simulink model "USV_MultiWaypoints"  (R2026b)
settings: Solver=VariableStepAuto  StopTime=300
undefined symbols (not defined in the file): arrival_dwell_time, arrival_radius, arrival_speed, current_bias_x, current_bias_y, current_change_time, current_estimation_tau, current_x, drag_r, drag_u, F_max, inertia_z, integral_activation_radius, K_aw, K_distance, Kd_heading, Ki_position, Ki_u, Kp_heading, Kp_u, M_max, mass_usv, position_integral_limit, u_max, wp1_x, wp1_y, wp2_x, wp2_y, wp3_x, wp3_y
libraries: simulink x1
settings Model: Creator=pablo  LastModifiedBy=pablo

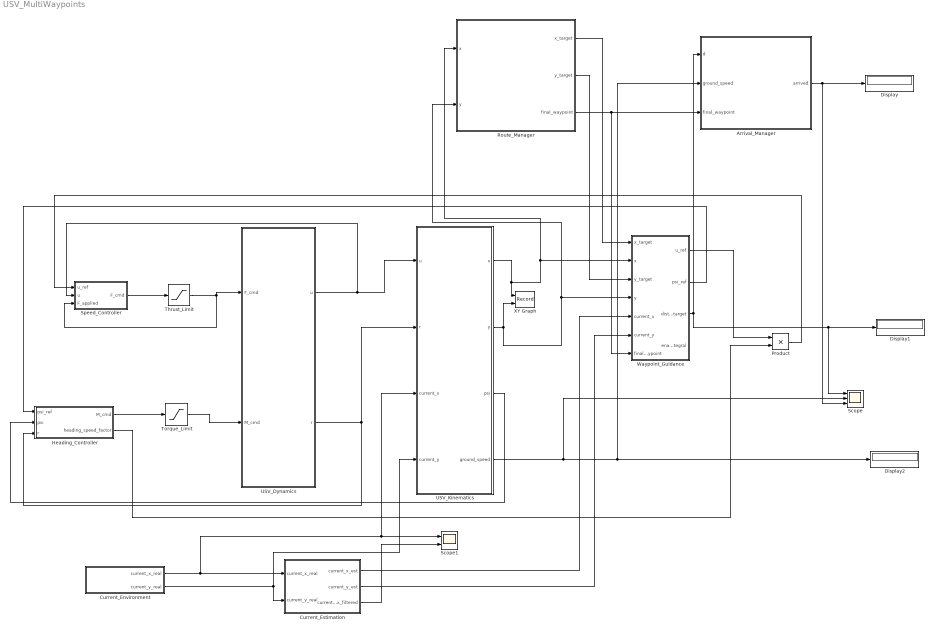
== system USV_MultiWaypoints ==
  Arrival_Manager : Stateflow chart  TreatAsAtomicUnit=on
  Current_Environment : Subsystem
  Current_Estimation : Subsystem
  Display : Display
  Display1 : Display
  Display2 : Display
  Heading_Controller : Subsystem
  Product : Product
  Route_Manager : Stateflow chart  TreatAsAtomicUnit=on
  Scope : Scope  NumInputPorts=3
      settings: ActiveDisplayYMinimum=-3.9141031212329302  ActiveDisplayYMaximum=39.009126348576444
  Scope1 : Scope  NumInputPorts=2
      settings: ActiveDisplayYMinimum=-0.25  ActiveDisplayYMaximum=0.25
  Speed_Controller : Subsystem
  Thrust_Limit : Saturate  UpperLimit=F_max  LowerLimit=-F_max
  Torque_Limit : Saturate  UpperLimit=M_max  LowerLimit=-M_max
  USV_Dynamics : Subsystem
  USV_Kinematics : Subsystem
  Waypoint_Guidance : Subsystem
  XY Graph : Record  NumPorts=2.0  FileSettingsInternal="{\"entries\":[{\"content\":{\"excelSettings\":{\"content\":{},\"type\":\"Streamout.ExcelSettings\"},\"parquetSettings\":{\"content\":{},\"type\":\"Streamout.ParquetSettings\"}},\"type\":\"Streamout.FileSettingStorage\",\"uuid\":\"\"}],\"packageUris\":[\"http:\\/\\/schema.mathworks.com\\/mf0\\/streamout_blocks\\/R2020a\"],\"version\":\"1.0\"}"  FrameSettings=[0, 0]  Layout=[1 1]  SignalsInternal="{\"entries\":[{\"content\":{\"signals\":[{\"content\":{\"blockPath\":[],\"dimensions\":[1],\"domain\":\"\",\"lineColor\":\"#a2142f\",\"plots\":[ 1 ],\"port\":1,\"sid\":[\"\"],\"signalID\":1,\"signalName\":\"USV_Kinematics:1\"},\"type\":\"RecordBlkView.Signal\",\"uuid\":\"\"},{\"content\":{\"blockPath\":[],\"dimensions\":[1],\"domain\":\"\",\"lineColor\":\"#139fff\",\"plots\":[ 1 ],\"port\":2,\"sid\":[\"\"],\"signalID\":2,\"signalName\":\"USV_Kinematics:2\"},\"type\":\"RecordBlkView.Signal\",\"uuid\":\"\"}]},\"type\":\"RecordBlkView.InputSignals\",\"uuid\":\"\"}],\"packageUris\":[\"http:\\/\\/schema.mathworks.com\\/mf0\\/streamout_blocks\\/R2020a\"],\"version\":\"1.0\"}"  VisualizationBindings="{\"xyplotplugin\":{\"info\":[{\"series\":[{\"bindingParametersList\":[{\"parameter\":\"X-Axis\",\"signalID\":1,\"signalName\":\"USV_Kinematics:1\"},{\"parameter\":\"Y-Axis\",\"signalID\":2,\"signalName\":\"USV_Kinematics:2\"}],\"seriesID\":0}],\"subplotID\":1}]}}"  CompatibilityTag=XY
  wires:
  USV_Dynamics/1(u) -> Speed_Controller/2(u), USV_Kinematics/1(u)
  USV_Dynamics/2(r) -> Heading_Controller/3(r), USV_Kinematics/2(r)
  Speed_Controller/1(F_cmd) -> Thrust_Limit/1
  Heading_Controller/1(M_cmd) -> Torque_Limit/1
  USV_Kinematics/3(psi) -> Heading_Controller/2(psi)
  USV_Kinematics/1(x) -> XY Graph/1, Route_Manager/1(x), Waypoint_Guidance/2(x)
  USV_Kinematics/2(y) -> Route_Manager/2(y), Waypoint_Guidance/4(y), XY Graph/2
  Waypoint_Guidance/2(psi_ref) -> Heading_Controller/1(psi_ref)
  Waypoint_Guidance/1(u_ref) -> Product/1
  Arrival_Manager/1(arrived) -> Scope/3, Display/1
  Waypoint_Guidance/3(distance_to_target) -> Arrival_Manager/1(d), Scope/1, Display1/1
  Route_Manager/1(x_target) -> Waypoint_Guidance/1(x_target)
  Route_Manager/2(y_target) -> Waypoint_Guidance/3(y_target)
  Route_Manager/3(final_waypoint) -> Waypoint_Guidance/7(final_waypoint), Arrival_Manager/3(final_waypoint)
  Thrust_Limit/1 -> USV_Dynamics/1(F_cmd), Speed_Controller/3(F_applied)
  Torque_Limit/1 -> USV_Dynamics/2(M_cmd)
  Heading_Controller/2(heading_speed_factor) -> Product/2
  Product/1 -> Speed_Controller/1(u_ref)
  USV_Kinematics/4(ground_speed) -> Scope/2, Arrival_Manager/2(ground_speed), Display2/1
  Current_Estimation/1(current_x_est) -> Waypoint_Guidance/5(current_x)
  Current_Estimation/2(current_y_est) -> Waypoint_Guidance/6(current_y)
  Current_Estimation/3(current_x_filtered) -> Scope1/2
  Current_Environment/1(current_x_real) -> Scope1/1, USV_Kinematics/3(current_x), Current_Estimation/1(current_x_real)
  Current_Environment/2(current_y_real) -> Current_Estimation/2(current_y_real), USV_Kinematics/4(current_y)

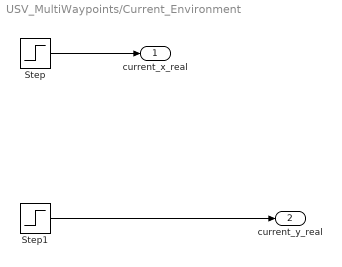
== system USV_MultiWaypoints/Current_Environment ==
  Step : Step  Time=current_change_time  InitialValue=current_x  FinalValue=current_x_after  SampleTime=0
  Step1 : Step  Time=current_change_time  InitialValue=current_y  FinalValue=current_y_after  SampleTime=0
  current_x_real : Outport
  current_y_real : Outport  Port=2
  wires:
  Step/1 -> current_x_real/1
  Step1/1 -> current_y_real/1

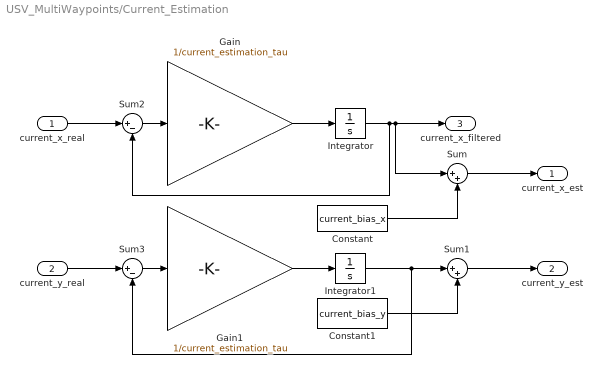
== system USV_MultiWaypoints/Current_Estimation ==
  current_x_real : Inport
  current_y_real : Inport  Port=2
  Constant : Constant  Value=current_bias_x
  Constant1 : Constant  Value=current_bias_y
  Gain : Gain  Gain=1/current_estimation_tau
  Gain1 : Gain  Gain=1/current_estimation_tau
  Integrator : Integrator  InitialCondition=current_x
  Integrator1 : Integrator  InitialCondition=current_x
  Sum : Sum  Inputs=|++
  Sum1 : Sum  Inputs=|++
  Sum2 : Sum  Inputs=|+-
  Sum3 : Sum  Inputs=|+-
  current_x_est : Outport
  current_y_est : Outport  Port=2
  current_x_filtered : Outport  Port=3
  wires:
  current_y_real/1 -> Sum3/1
  current_x_real/1 -> Sum2/1
  Gain1/1 -> Integrator1/1
  Sum2/1 -> Gain/1
  Sum3/1 -> Gain1/1
  Gain/1 -> Integrator/1
  Integrator/1 -> Sum/1, current_x_filtered/1, Sum2/2
  Constant/1 -> Sum/2
  Integrator1/1 -> Sum3/2, Sum1/1
  Constant1/1 -> Sum1/2
  Sum/1 -> current_x_est/1
  Sum1/1 -> current_y_est/1

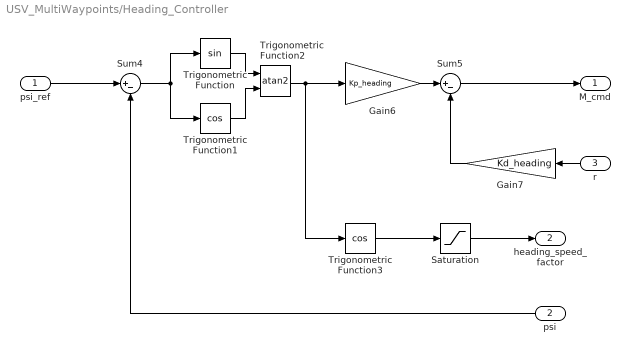
== system USV_MultiWaypoints/Heading_Controller ==
  psi_ref : Inport
  psi : Inport  Port=2
  r : Inport  Port=3
  Gain6 : Gain  Gain=Kp_heading
  Gain7 : Gain  Gain=Kd_heading
  Saturation : Saturate  UpperLimit=1  LowerLimit=0
  Sum4 : Sum  Inputs=|+-
  Sum5 : Sum  Inputs=|+-
  Trigonometric Function : Trigonometry
  Trigonometric Function1 : Trigonometry  Operator=cos
  Trigonometric Function2 : Trigonometry  Operator=atan2
  Trigonometric Function3 : Trigonometry  Operator=cos
  M_cmd : Outport
  heading_speed_factor : Outport  Port=2
  wires:
  Sum5/1 -> M_cmd/1
  psi_ref/1 -> Sum4/1
  r/1 -> Gain7/1
  Gain6/1 -> Sum5/1
  psi/1 -> Sum4/2
  Gain7/1 -> Sum5/2
  Sum4/1 -> Trigonometric Function/1, Trigonometric Function1/1
  Trigonometric Function/1 -> Trigonometric Function2/1
  Trigonometric Function1/1 -> Trigonometric Function2/2
  Trigonometric Function2/1 -> Trigonometric Function3/1, Gain6/1
  Trigonometric Function3/1 -> Saturation/1
  Saturation/1 -> heading_speed_factor/1

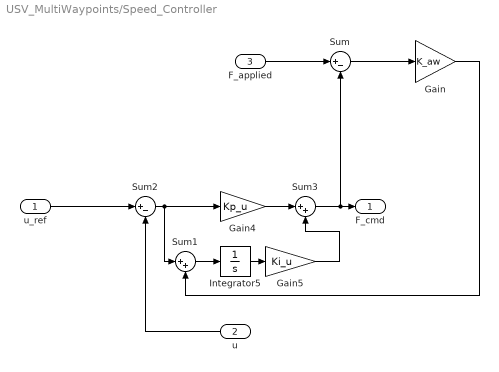
== system USV_MultiWaypoints/Speed_Controller ==
  u_ref : Inport
  u : Inport  Port=2
  F_applied : Inport  Port=3
  Gain : Gain  Gain=K_aw
  Gain4 : Gain  Gain=Kp_u
  Gain5 : Gain  Gain=Ki_u
  Integrator5 : Integrator
  Sum : Sum  Inputs=|+-
  Sum1 : Sum  Inputs=|++
  Sum2 : Sum  Inputs=|+-
  Sum3 : Sum  Inputs=|++
  F_cmd : Outport
  wires:
  Integrator5/1 -> Gain5/1
  u_ref/1 -> Sum2/1
  u/1 -> Sum2/2
  Gain5/1 -> Sum3/2
  Sum2/1 -> Sum1/1, Gain4/1
  Gain4/1 -> Sum3/1
  Sum3/1 -> Sum/2, F_cmd/1
  F_applied/1 -> Sum/1
  Sum/1 -> Gain/1
  Sum1/1 -> Integrator5/1
  Gain/1 -> Sum1/2

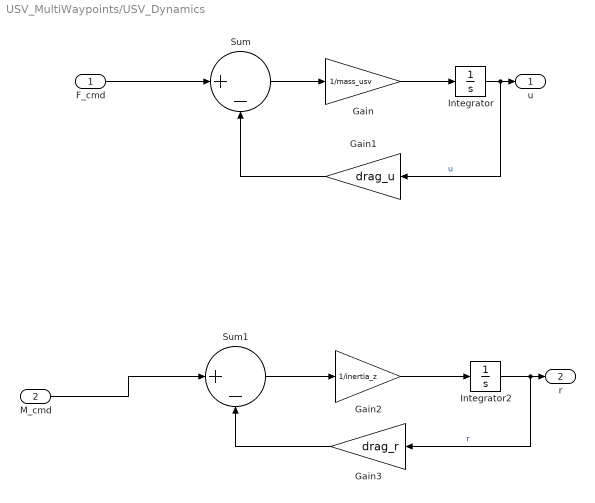
== system USV_MultiWaypoints/USV_Dynamics ==
  F_cmd : Inport
  M_cmd : Inport  Port=2
  Gain : Gain  Gain=1/mass_usv
  Gain1 : Gain  Gain=drag_u
  Gain2 : Gain  Gain=1/inertia_z
  Gain3 : Gain  Gain=drag_r
  Integrator : Integrator
  Integrator2 : Integrator
  Sum : Sum  Inputs=|+-
  Sum1 : Sum  Inputs=|+-
  u : Outport
  r : Outport  Port=2
  wires:
  F_cmd/1 -> Sum/1
  Gain2/1 -> Integrator2/1
  Gain3/1 -> Sum1/2
  Integrator/1 -> Gain1/1, u/1  "u"
  Sum/1 -> Gain/1
  Gain/1 -> Integrator/1
  Gain1/1 -> Sum/2
  Sum1/1 -> Gain2/1
  Integrator2/1 -> Gain3/1, r/1  "r"
  M_cmd/1 -> Sum1/1

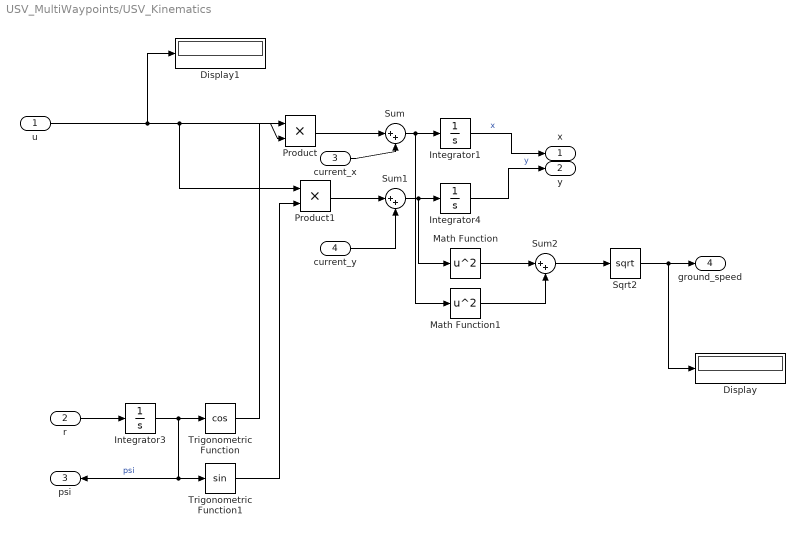
== system USV_MultiWaypoints/USV_Kinematics ==
  u : Inport
  r : Inport  Port=2
  current_x : Inport  Port=3
  current_y : Inport  Port=4
  Display : Display
  Display1 : Display
  Integrator1 : Integrator
  Integrator3 : Integrator
  Integrator4 : Integrator
  Math Function : Math  Operator=square
  Math Function1 : Math  Operator=square
  Product : Product
  Product1 : Product
  Sqrt2 : Sqrt
  Sum : Sum  Inputs=|++
  Sum1 : Sum  Inputs=|++
  Sum2 : Sum  Inputs=|++
  Trigonometric Function : Trigonometry  Operator=cos
  Trigonometric Function1 : Trigonometry
  x : Outport
  y : Outport  Port=2
  psi : Outport  Port=3
  ground_speed : Outport  Port=4
  wires:
  Integrator3/1 -> Trigonometric Function1/1, psi/1, Trigonometric Function/1  "psi"
  Trigonometric Function/1 -> Product/1
  u/1 -> Display1/1, Product1/1, Product/2
  Product/1 -> Sum/1
  Product1/1 -> Sum1/1
  r/1 -> Integrator3/1
  Trigonometric Function1/1 -> Product1/2
  Integrator1/1 -> x/1  "x"
  Integrator4/1 -> y/1  "y"
  current_y/1 -> Sum1/2
  current_x/1 -> Sum/2
  Sum/1 -> Math Function1/1, Integrator1/1
  Sum1/1 -> Math Function/1, Integrator4/1
  Math Function/1 -> Sum2/1
  Math Function1/1 -> Sum2/2
  Sum2/1 -> Sqrt2/1
  Sqrt2/1 -> Display/1, ground_speed/1

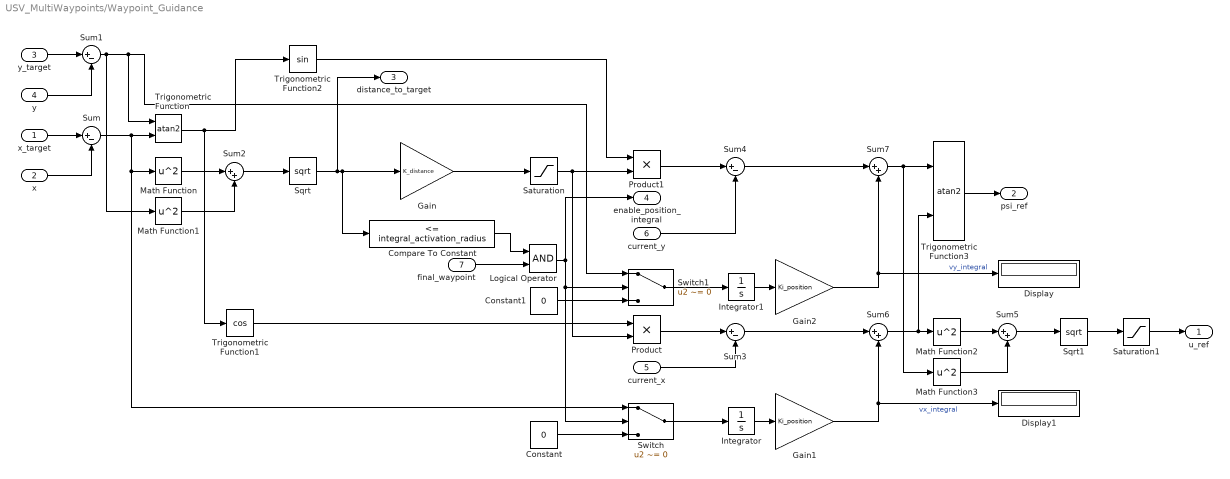
== system USV_MultiWaypoints/Waypoint_Guidance ==
  x_target : Inport
  x : Inport  Port=2
  y_target : Inport  Port=3
  y : Inport  Port=4
  current_x : Inport  Port=5
  current_y : Inport  Port=6
  final_waypoint : Inport  Port=7
  Compare To Constant : simulink/Logic and Bit Operations/Compare To Constant  relop=<=  const=integral_activation_radius  OutDataTypeStr=boolean
  Constant : Constant  Value=0
  Constant1 : Constant  Value=0
  Display : Display
  Display1 : Display
  Gain : Gain  Gain=K_distance
  Gain1 : Gain  Gain=Ki_position
  Gain2 : Gain  Gain=Ki_position
  Integrator : Integrator  LimitOutput=on  UpperSaturationLimit=position_integral_limit  LowerSaturationLimit=-position_integral_limit
  Integrator1 : Integrator  LimitOutput=on  UpperSaturationLimit=position_integral_limit  LowerSaturationLimit=-position_integral_limit
  Logical Operator : Logic  AllPortsSameDT=off  OutDataTypeStr=boolean
  Math Function{,1..3} (4 alike) : Math  Operator=square
  Product : Product
  Product1 : Product
  Saturation : Saturate  UpperLimit=u_max  LowerLimit=0
  Saturation1 : Saturate  UpperLimit=u_max  LowerLimit=0
  Sqrt : Sqrt
  Sqrt1 : Sqrt
  Sum{,1,3..4} (4 alike) : Sum  Inputs=|+-
  Sum{2,5..7} (4 alike) : Sum  Inputs=|++
  Switch : Switch  Criteria=u2 ~= 0  SaturateOnIntegerOverflow=off  InputSameDT=off
  Switch1 : Switch  Criteria=u2 ~= 0  SaturateOnIntegerOverflow=off  InputSameDT=off
  Trigonometric Function : Trigonometry  Operator=atan2
  Trigonometric Function1 : Trigonometry  Operator=cos
  Trigonometric Function2 : Trigonometry
  Trigonometric Function3 : Trigonometry  Operator=atan2
  u_ref : Outport
  psi_ref : Outport  Port=2
  distance_to_target : Outport  Port=3
  enable_position_integral : Outport  Port=4
  wires:
  Product/1 -> Sum3/1
  current_y/1 -> Sum4/2
  x/1 -> Sum/2
  x_target/1 -> Sum/1
  Product1/1 -> Sum4/1
  y/1 -> Sum1/2
  y_target/1 -> Sum1/1
  Switch1/1 -> Integrator1/1
  Trigonometric Function/1 -> Trigonometric Function2/1, Trigonometric Function1/1
  Math Function/1 -> Sum2/1
  Math Function2/1 -> Sum5/1
  Sum2/1 -> Sqrt/1
  Sum/1 -> Switch/1, Math Function/1, Trigonometric Function/2
  Sqrt/1 -> Gain/1, Compare To Constant/1, distance_to_target/1
  Sum1/1 -> Switch1/1, Trigonometric Function/1, Math Function1/1
  Saturation1/1 -> u_ref/1
  Math Function1/1 -> Sum2/2
  Trigonometric Function1/1 -> Product/1
  Switch/1 -> Integrator/1
  Trigonometric Function2/1 -> Product1/1
  Gain/1 -> Saturation/1
  Compare To Constant/1 -> Logical Operator/1
  final_waypoint/1 -> Logical Operator/2
  Constant/1 -> Switch/3
  Saturation/1 -> Product/2, Product1/2
  Sum4/1 -> Sum7/1
  Logical Operator/1 -> Switch/2, Switch1/2, enable_position_integral/1
  Sum6/1 -> Math Function2/1, Trigonometric Function3/2
  Constant1/1 -> Switch1/3
  current_x/1 -> Sum3/2
  Integrator1/1 -> Gain2/1
  Sum3/1 -> Sum6/1
  Integrator/1 -> Gain1/1
  Gain2/1 -> Sum7/2, Display/1  "vy_integral"
  Gain1/1 -> Display1/1, Sum6/2  "vx_integral"
  Sum7/1 -> Math Function3/1, Trigonometric Function3/1
  Trigonometric Function3/1 -> psi_ref/1
  Sum5/1 -> Sqrt1/1
  Math Function3/1 -> Sum5/2
  Sqrt1/1 -> Saturation1/1

== stateflow chart USV_MultiWaypoints/Route_Manager ==
  state Waypoint_1
    entry:
    x_target = wp1_x;
    y_target = wp1_y;
    final_waypoint = 0;
  state Waypoint_2
    entry:
    x_target = wp2_x;
    y_target = wp2_y;
    final_waypoint = 0;
  state Waypoint_3
    entry:
    x_target = wp3_x;
    y_target = wp3_y;
    final_waypoint = 1;
  (default) -> Waypoint_1
  Waypoint_1 -> Waypoint_2 : [(x-wp1_x)^2 + (y-wp1_y)^2 <= arrival_radius^2]
  Waypoint_2 -> Waypoint_3 : [(x-wp2_x)^2 + (y-wp2_y)^2 <= arrival_radius^2]
  data: x input; y input; x_target output; y_target output; final_waypoint output; arrival_radius parameter; wp3_y parameter; wp3_x parameter; wp2_y parameter; wp2_x parameter; wp1_y parameter; wp1_x parameter

== stateflow chart USV_MultiWaypoints/Arrival_Manager ==
  state Navigating
    entry:
    arrived = 0;
  state Settling
    entry:
    arrived = 0;
  state Confirming
    entry:
    arrived = 0;
  state Arrived
    entry:
    arrived = 1;
  (default) -> Navigating
  Navigating -> Settling : [final_waypoint == 1 && d <= arrival_radius]
  Arrived -> Settling : [d > 2*arrival_radius || ground_speed > 2*arrival_speed]
  Confirming -> Settling [order 1] : [d > arrival_radius || ground_speed > arrival_speed]
  Settling -> Confirming : [d <= arrival_radius && ground_speed <= arrival_speed]
  Confirming -> Arrived [order 2] : [after(arrival_dwell_time, sec) && d <= arrival_radius && ground_speed <= arrival_speed]
  data: d input; ground_speed input; arrived output; final_waypoint input; arrival_speed parameter; arrival_radius parameter; arrival_dwell_time parameter
